simulink model "simPmatrixTest"  (R2020a)
settings: Solver=VariableStepAuto  StartTime=0.0  StopTime=10.0  RelTol=1e-3
undefined symbols (not defined in the file or in its folder): preal
libraries: lpvcoreLibraryCore x3
settings Model: Creator=Patrick  LastModifiedBy=Patrick
settings DataIOCC: SaveOutput=off  SignalLogging=off  DSMLogging=off  SaveTime=off

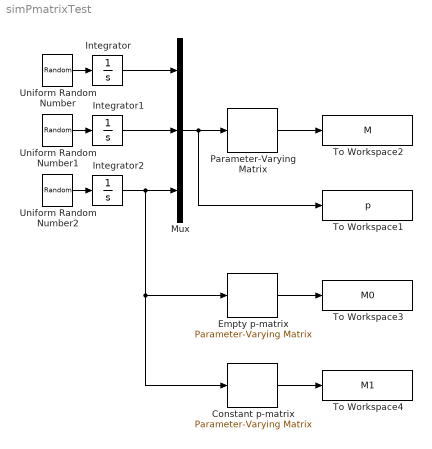
== system simPmatrixTest ==
  Constant p-matrix : lpvcoreLibraryCore/Parameter-Varying Matrix  M=0*preal('p')+2
      settings: SourceProductName=LPVcore
  Empty p-matrix : lpvcoreLibraryCore/Parameter-Varying Matrix  M=[]*preal('p','dt')
      settings: SourceProductName=LPVcore
  Integrator : Integrator
  Integrator1 : Integrator
  Integrator2 : Integrator
  Mux : Mux  Inputs=3
  Parameter-Varying Matrix : lpvcoreLibraryCore/Parameter-Varying Matrix  M=Mp
      settings: SourceProductName=LPVcore
  To Workspace1 : ToWorkspace  VariableName=p  SampleTime=-1
  To Workspace2 : ToWorkspace  VariableName=M  SampleTime=-1
  To Workspace3 : ToWorkspace  VariableName=M0  SampleTime=-1
  To Workspace4 : ToWorkspace  VariableName=M1  SampleTime=-1
  Uniform Random Number : UniformRandomNumber  SampleTime=0.1
  Uniform Random Number1 : UniformRandomNumber  Seed=1  SampleTime=0.1
  Uniform Random Number2 : UniformRandomNumber  Seed=2  SampleTime=0.1
  wires:
  Uniform Random Number/1 -> Integrator/1
  Parameter-Varying Matrix/1 -> To Workspace2/1
  Uniform Random Number1/1 -> Integrator1/1
  Uniform Random Number2/1 -> Integrator2/1
  Integrator1/1 -> Mux/2
  Integrator/1 -> Mux/1
  Mux/1 -> To Workspace1/1, Parameter-Varying Matrix/1
  Empty p-matrix/1 -> To Workspace3/1
  Integrator2/1 -> Constant p-matrix/1, Empty p-matrix/1, Mux/3
  Constant p-matrix/1 -> To Workspace4/1
